simulink model "BESS_PV_WIND_STAGE2_R1_with_scopes"  (R2024b)
settings: Solver=VariableStepAuto  StartTime=0.0  StopTime=10.0  RelTol=1e-3
InitFcn:
  | run(fullfile(fileparts(get_param(bdroot,'FileName')),'..','scripts','init_bess_pv_wind_stage2_r1.m'));
undefined symbols (not defined in the file): Control, G, S1, S2, S21, W1
libraries: ee_lib x27, nesl_utility x23, fl_lib x10, simulink x5
(part 2 of 2)

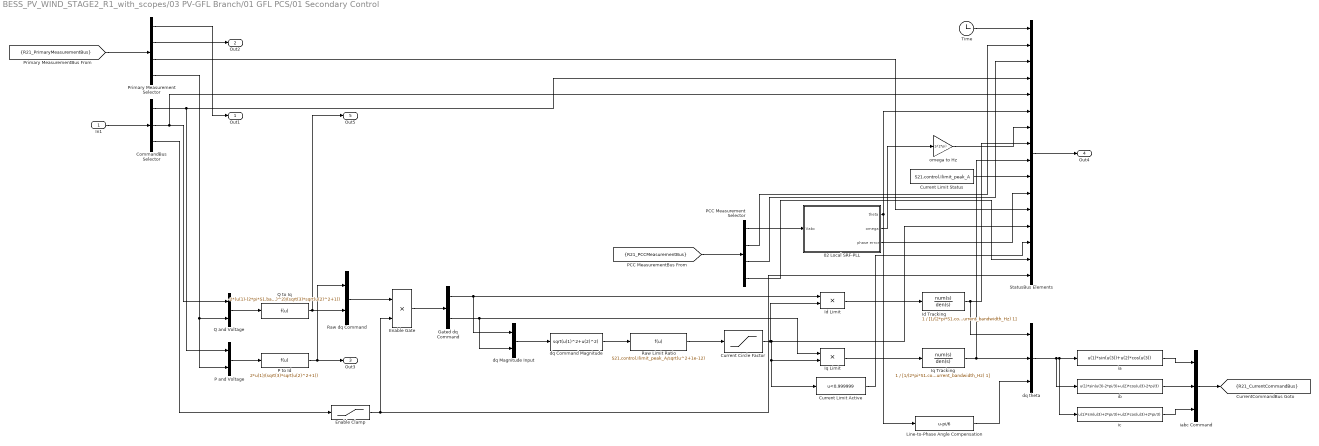
== system BESS_PV_WIND_STAGE2_R1_with_scopes/03 PV-GFL Branch/01 GFL PCS/01 Secondary Control ==
  In1 : Inport
  02 Local SRF-PLL : Subsystem
      settings: AttributesFormatString=|
      | local abc voltage only
      | wrapped phase-error PI
  CommandBus Selector : Demux  Outputs=3
  Current Circle Factor : Saturate  UpperLimit=1  LowerLimit=0
  Current Limit Active : Fcn  Expr=u<0.999999
  Current Limit Status : Constant  Value=S21.control.Ilimit_peak_A
  Enable Clamp : Saturate  UpperLimit=1  LowerLimit=0
  Enable Gate : Product  Inputs=**
  Gated dq Command : Demux  Outputs=2
  Id Limit : Product  Inputs=**
  Id Tracking : TransferFcn  Numerator=1  Denominator=[1/(2*pi*S1.control.current_bandwidth_Hz) 1]
  Iq Limit : Product  Inputs=**
  Iq Tracking : TransferFcn  Numerator=1  Denominator=[1/(2*pi*S1.control.current_bandwidth_Hz) 1]
  Line-to-Phase Angle Compensation : Fcn  Expr=u-pi/6
  P and Voltage : Mux  Inputs=2
  P to Id : Fcn  Expr=2*u(1)/(sqrt(3)*sqrt(u(2)^2+1))
  PCC Measurement Selector : Demux  Outputs=[3 1 1 1]
  Primary Measurement Selector : Demux  Outputs=[3 3 1 1]
  Q and Voltage : Mux  Inputs=2
  Q to Iq : Fcn  Expr=-2*(u(1)-(2*pi*S1.base.f_Hz*S1.filter.C_F/2)*u(2)^2)/(sqrt(3)*sqrt(u(2)^2+1))
  Raw Limit Ratio : Fcn  Expr=S21.control.Ilimit_peak_A/sqrt(u^2+1e-12)
  Raw dq Command : Mux  Inputs=2
  StatusBus Elements : Mux  Inputs=16
  Time : Clock
  dq Command Magnitude : Fcn  Expr=sqrt(u(1)^2+u(2)^2)
  dq Magnitude Input : Mux  Inputs=2
  dq theta : Mux  Inputs=3
  ia : Fcn  Expr=u(1)*sin(u(3))+u(2)*cos(u(3))
  iabc Command : Mux  Inputs=3
  ib : Fcn  Expr=u(1)*sin(u(3)-2*pi/3)+u(2)*cos(u(3)-2*pi/3)
  ic : Fcn  Expr=u(1)*sin(u(3)+2*pi/3)+u(2)*cos(u(3)+2*pi/3)
  omega to Hz : Gain  Gain=1/(2*pi)
  Out1 : Outport
  Out2 : Outport  Port=2
  Out3 : Outport  Port=3
  Out4 : Outport  Port=4
  Out5 : Outport  Port=5
  tag scope: R21_CurrentCommandBus=scoped
  wires:
  PCC Measurement Selector/4 -> StatusBus Elements/15
  Q and Voltage/1 -> Q to Iq/1
  Primary Measurement Selector/4 -> Q and Voltage/2, P and Voltage/2
  PCC Measurement Selector/3 -> StatusBus Elements/3
  Primary Measurement Selector/3 -> StatusBus Elements/12
  PCC Measurement Selector/2 -> StatusBus Elements/2
  Primary Measurement Selector/2 -> Out2/1
  PCC Measurement Selector/1 -> 02 Local SRF-PLL/1(Vabc)
  Primary Measurement Selector/1 -> Out1/1
  [R21_PCCMeasurementBus] -> PCC Measurement Selector/1
  Raw dq Command/1 -> Enable Gate/1
  [R21_PrimaryMeasurementBus] -> Primary Measurement Selector/1
  In1/1 -> CommandBus Selector/1
  CommandBus Selector/2 -> StatusBus Elements/5, Q and Voltage/1
  Current Limit Active/1 -> StatusBus Elements/14
  CommandBus Selector/1 -> P and Voltage/1, StatusBus Elements/4
  Current Limit Status/1 -> StatusBus Elements/10
  CommandBus Selector/3 -> Enable Clamp/1
  Id Tracking/1 -> StatusBus Elements/8, dq theta/1
  Gated dq Command/1 -> Id Limit/1, dq Magnitude Input/1
  P and Voltage/1 -> P to Id/1
  Q to Iq/1 -> Raw dq Command/2, Out5/1
  Gated dq Command/2 -> Iq Limit/1, dq Magnitude Input/2
  P to Id/1 -> Raw dq Command/1, Out3/1
  Enable Clamp/1 -> StatusBus Elements/16, Enable Gate/2
  Id Limit/1 -> Id Tracking/1
  Enable Gate/1 -> Gated dq Command/1
  dq Magnitude Input/1 -> dq Command Magnitude/1
  dq Command Magnitude/1 -> Raw Limit Ratio/1
  Raw Limit Ratio/1 -> Current Circle Factor/1
  Current Circle Factor/1 -> Current Limit Active/1, Iq Limit/2, StatusBus Elements/13, Id Limit/2
  02 Local SRF-PLL/1(theta) -> StatusBus Elements/6, Line-to-Phase Angle Compensation/1
  02 Local SRF-PLL/2(omega) -> omega to Hz/1
  02 Local SRF-PLL/3(phase error) -> StatusBus Elements/11
  Iq Limit/1 -> Iq Tracking/1
  Time/1 -> StatusBus Elements/1
  dq theta/1 -> ic/1, ia/1, ib/1
  omega to Hz/1 -> StatusBus Elements/7
  Iq Tracking/1 -> StatusBus Elements/9, dq theta/2
  Line-to-Phase Angle Compensation/1 -> dq theta/3
  StatusBus Elements/1 -> Out4/1
  ia/1 -> iabc Command/1
  ib/1 -> iabc Command/2
  ic/1 -> iabc Command/3
  iabc Command/1 -> [R21_CurrentCommandBus]

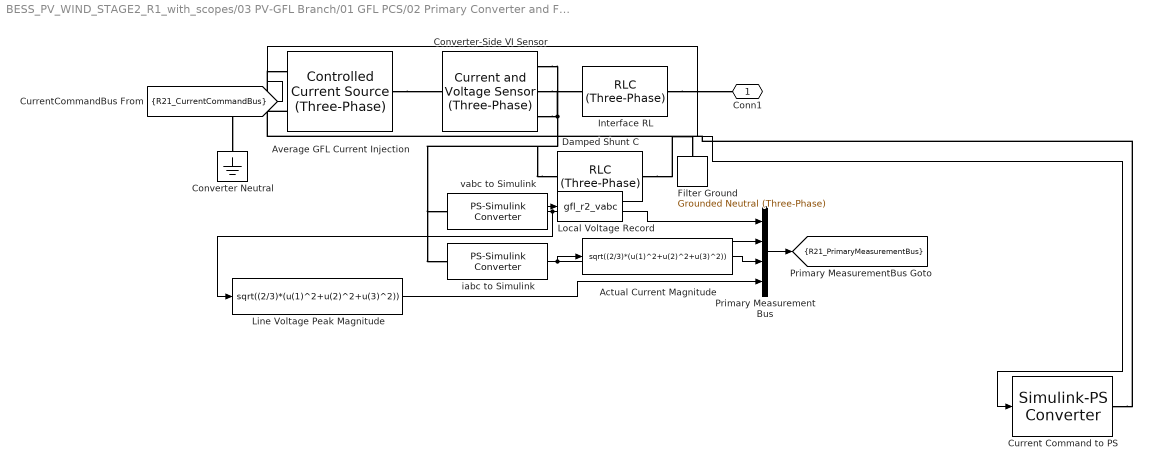
== system BESS_PV_WIND_STAGE2_R1_with_scopes/03 PV-GFL Branch/01 GFL PCS/02 Primary Converter and Filter ==
  Actual Current Magnitude : Fcn  Expr=sqrt((2/3)*(u(1)^2+u(2)^2+u(3)^2))
  Average GFL Current Injection : ee_lib/Sources/Controlled Current Source (Three-Phase)  port_option=ee.enum.threePhasePort.composite  input_option=ee.enum.inputType.instantaneous  FRated=S1.base.f_Hz Hz  G_parasitic=1e-6 1/Ohm
  Converter Neutral : fl_lib/Electrical/Electrical Elements/Electrical Reference
  Converter-Side VI Sensor : ee_lib/Sensors & Transducers/Current and Voltage Sensor (Three-Phase)  port_option=ee.enum.threePhasePort.composite  vMeasurementType=ee.enum.vmeasurement.ll  outputUnit=ee.enum.unit.si  SRated=100e6 A*V  VRated=24e3 V  I_specify=off  I_priority=None  I=[0, 0, 0] A  I_nominal_specify=off  I_nominal_value=1  I_nominal_unit=A  V_specify=off  V_priority=None  V=[0, 0, 0] V  V_nominal_specify=off  V_nominal_value=1  V_nominal_unit=V
  Current Command to PS : nesl_utility/Simulink-PS Converter  PhysicalDomain=network_engine_domain  SubClassName=ps_input  LeftPortType=input  RightPortType=output  PseudoPeriodic=off  Frequencies=[]  NoiseDistribution=none  NoiseParameters=[]  Unit=A  AffineConversion=off  FilteringAndDerivatives=zero  SimscapeFilterOrder=1  InputFilterTimeConstant=0.001  UdotUserProvided=0
  Damped Shunt C : ee_lib/Passive/RLC Assemblies/RLC (Three-Phase)  port_option=ee.enum.threePhasePort.composite  component_structure=ee.enum.rlc.structure.SeriesRC  R=S1.filter.Rd_ohm Ohm  L=1e-3 H  C=S1.filter.C_F F  R_parasitic=0 Ohm  G_parasitic=0 1/Ohm  IL_specify=off  IL_priority=High  IL=[0, 0, 0] A  IL_nominal_specify=off  IL_nominal_value=1  IL_nominal_unit=A  VC_specify=off  VC_priority=High  VC=[0, 0, 0] V  VC_nominal_specify=off  VC_nominal_value=1  VC_nominal_unit=V
  Filter Ground : ee_lib/Connectors & References/Grounded Neutral (Three-Phase)  port_option=ee.enum.threePhasePort.composite
  Interface RL : ee_lib/Passive/RLC Assemblies/RLC (Three-Phase)  port_option=ee.enum.threePhasePort.composite  component_structure=ee.enum.rlc.structure.R  R=S1.filter.R1_ohm+S1.filter.R2_ohm Ohm  L=1e-3 H  C=1e-6 F  R_parasitic=0 Ohm  G_parasitic=0 1/Ohm  IL_specify=off  IL_priority=High  IL=[0, 0, 0] A  IL_nominal_specify=off  IL_nominal_value=1  IL_nominal_unit=A  VC_specify=off  VC_priority=High  VC=[0, 0, 0] V  VC_nominal_specify=off  VC_nominal_value=1  VC_nominal_unit=V
  Line Voltage Peak Magnitude : Fcn  Expr=sqrt((2/3)*(u(1)^2+u(2)^2+u(3)^2))
  Local Voltage Record : ToWorkspace  VariableName=gfl_r2_vabc  SampleTime=-1
  Primary MeasurementBus : Mux
  iabc to Simulink : nesl_utility/PS-Simulink Converter  PhysicalDomain=network_engine_domain  SubClassName=ps_output  LeftPortType=input  RightPortType=output  PseudoPeriodic=off  Frequencies=[]  VectorFormat=inherit  Unit=A  AffineConversion=off
  vabc to Simulink : nesl_utility/PS-Simulink Converter  PhysicalDomain=network_engine_domain  SubClassName=ps_output  LeftPortType=input  RightPortType=output  PseudoPeriodic=off  Frequencies=[]  VectorFormat=inherit  Unit=V  AffineConversion=off
  Conn1 : PMIOPort  Side=Right
  tag scope: R21_PrimaryMeasurementBus=scoped
  wires:
  iabc to Simulink/1 -> Primary MeasurementBus/2, Actual Current Magnitude/1
  vabc to Simulink/1 -> Primary MeasurementBus/1, Line Voltage Peak Magnitude/1, Local Voltage Record/1
  [R21_CurrentCommandBus] -> Current Command to PS/1
  Primary MeasurementBus/1 -> [R21_PrimaryMeasurementBus]
  Actual Current Magnitude/1 -> Primary MeasurementBus/3
  Line Voltage Peak Magnitude/1 -> Primary MeasurementBus/4
  connections:
  Damped Shunt C/LConn1 -- Converter-Side VI Sensor/RConn3 -- Interface RL/LConn1
  Current Command to PS/RConn1 -- Average GFL Current Injection/LConn1
  Converter-Side VI Sensor/RConn1 -- vabc to Simulink/LConn1
  Average GFL Current Injection/LConn2 -- Converter Neutral/LConn1
  Interface RL/RConn1 -- Conn1/RConn1
  Converter-Side VI Sensor/RConn2 -- iabc to Simulink/LConn1
  Damped Shunt C/RConn1 -- Filter Ground/LConn1
  Average GFL Current Injection/RConn1 -- Converter-Side VI Sensor/LConn1

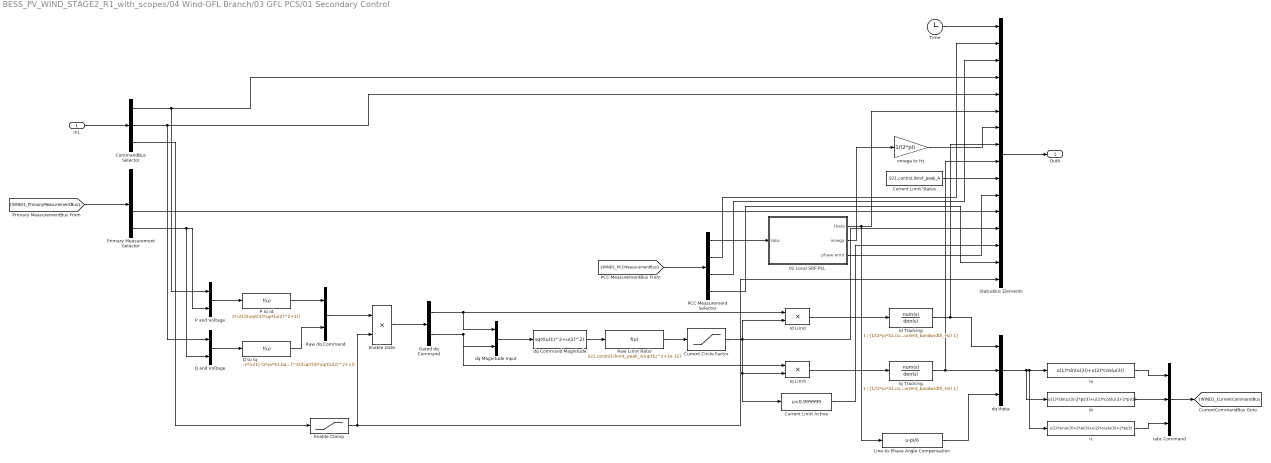
== system BESS_PV_WIND_STAGE2_R1_with_scopes/04 Wind-GFL Branch/03 GFL PCS/01 Secondary Control ==
  In1 : Inport
  02 Local SRF-PLL : Subsystem
      settings: AttributesFormatString=|
      | local abc voltage only
      | wrapped phase-error PI
  CommandBus Selector : Demux  Outputs=3
  Current Circle Factor : Saturate  UpperLimit=1  LowerLimit=0
  Current Limit Active : Fcn  Expr=u<0.999999
  Current Limit Status : Constant  Value=S21.control.Ilimit_peak_A
  Enable Clamp : Saturate  UpperLimit=1  LowerLimit=0
  Enable Gate : Product  Inputs=**
  Gated dq Command : Demux  Outputs=2
  Id Limit : Product  Inputs=**
  Id Tracking : TransferFcn  Numerator=1  Denominator=[1/(2*pi*S1.control.current_bandwidth_Hz) 1]
  Iq Limit : Product  Inputs=**
  Iq Tracking : TransferFcn  Numerator=1  Denominator=[1/(2*pi*S1.control.current_bandwidth_Hz) 1]
  Line-to-Phase Angle Compensation : Fcn  Expr=u-pi/6
  P and Voltage : Mux  Inputs=2
  P to Id : Fcn  Expr=2*u(1)/(sqrt(3)*sqrt(u(2)^2+1))
  PCC Measurement Selector : Demux  Outputs=[3 1 1 1]
  Primary Measurement Selector : Demux  Outputs=[3 3 1 1]
  Q and Voltage : Mux  Inputs=2
  Q to Iq : Fcn  Expr=-2*(u(1)-(2*pi*S1.base.f_Hz*S1.filter.C_F/2)*u(2)^2)/(sqrt(3)*sqrt(u(2)^2+1))
  Raw Limit Ratio : Fcn  Expr=S21.control.Ilimit_peak_A/sqrt(u^2+1e-12)
  Raw dq Command : Mux  Inputs=2
  StatusBus Elements : Mux  Inputs=16
  Time : Clock
  dq Command Magnitude : Fcn  Expr=sqrt(u(1)^2+u(2)^2)
  dq Magnitude Input : Mux  Inputs=2
  dq theta : Mux  Inputs=3
  ia : Fcn  Expr=u(1)*sin(u(3))+u(2)*cos(u(3))
  iabc Command : Mux  Inputs=3
  ib : Fcn  Expr=u(1)*sin(u(3)-2*pi/3)+u(2)*cos(u(3)-2*pi/3)
  ic : Fcn  Expr=u(1)*sin(u(3)+2*pi/3)+u(2)*cos(u(3)+2*pi/3)
  omega to Hz : Gain  Gain=1/(2*pi)
  Out4 : Outport
  tag scope: WIND1_CurrentCommandBus=scoped
  wires:
  In1/1 -> CommandBus Selector/1
  Primary Measurement Selector/4 -> P and Voltage/2, Q and Voltage/2
  Enable Clamp/1 -> StatusBus Elements/16, Enable Gate/2
  P to Id/1 -> Raw dq Command/1
  [WIND1_PrimaryMeasurementBus] -> Primary Measurement Selector/1
  CommandBus Selector/3 -> Enable Clamp/1
  CommandBus Selector/1 -> StatusBus Elements/4, P and Voltage/1
  CommandBus Selector/2 -> StatusBus Elements/5, Q and Voltage/1
  Id Tracking/1 -> dq theta/1, StatusBus Elements/8
  P and Voltage/1 -> P to Id/1
  Primary Measurement Selector/3 -> StatusBus Elements/12
  Q and Voltage/1 -> Q to Iq/1
  iabc Command/1 -> [WIND1_CurrentCommandBus]
  Q to Iq/1 -> Raw dq Command/2
  Raw dq Command/1 -> Enable Gate/1
  PCC Measurement Selector/2 -> StatusBus Elements/2
  Enable Gate/1 -> Gated dq Command/1
  Gated dq Command/1 -> Id Limit/1, dq Magnitude Input/1
  [WIND1_PCCMeasurementBus] -> PCC Measurement Selector/1
  Gated dq Command/2 -> Iq Limit/1, dq Magnitude Input/2
  dq Magnitude Input/1 -> dq Command Magnitude/1
  dq Command Magnitude/1 -> Raw Limit Ratio/1
  Raw Limit Ratio/1 -> Current Circle Factor/1
  Iq Limit/1 -> Iq Tracking/1
  PCC Measurement Selector/1 -> 02 Local SRF-PLL/1(Vabc)
  PCC Measurement Selector/3 -> StatusBus Elements/3
  Iq Tracking/1 -> StatusBus Elements/9, dq theta/2
  Current Circle Factor/1 -> Current Limit Active/1, Iq Limit/2, StatusBus Elements/13, Id Limit/2
  PCC Measurement Selector/4 -> StatusBus Elements/15
  02 Local SRF-PLL/1(theta) -> StatusBus Elements/6, Line-to-Phase Angle Compensation/1
  02 Local SRF-PLL/2(omega) -> omega to Hz/1
  02 Local SRF-PLL/3(phase error) -> StatusBus Elements/11
  Id Limit/1 -> Id Tracking/1
  Line-to-Phase Angle Compensation/1 -> dq theta/3
  Current Limit Active/1 -> StatusBus Elements/14
  Time/1 -> StatusBus Elements/1
  dq theta/1 -> ia/1, ic/1, ib/1
  omega to Hz/1 -> StatusBus Elements/7
  Current Limit Status/1 -> StatusBus Elements/10
  StatusBus Elements/1 -> Out4/1
  ia/1 -> iabc Command/1
  ib/1 -> iabc Command/2
  ic/1 -> iabc Command/3

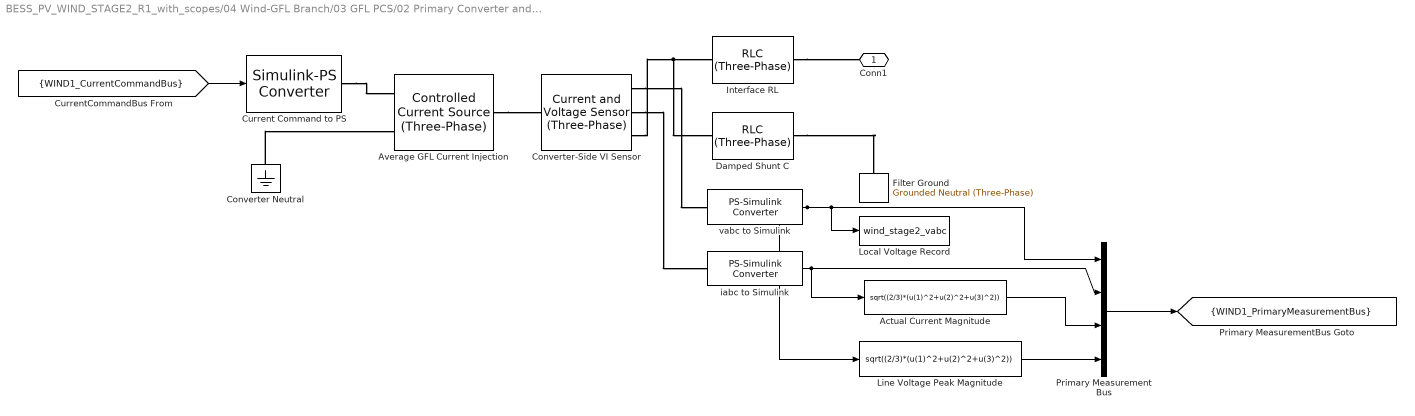
== system BESS_PV_WIND_STAGE2_R1_with_scopes/04 Wind-GFL Branch/03 GFL PCS/02 Primary Converter and Filter ==
  Actual Current Magnitude : Fcn  Expr=sqrt((2/3)*(u(1)^2+u(2)^2+u(3)^2))
  Average GFL Current Injection : ee_lib/Sources/Controlled Current Source (Three-Phase)  port_option=ee.enum.threePhasePort.composite  input_option=ee.enum.inputType.instantaneous  FRated=S1.base.f_Hz Hz  G_parasitic=1e-6 1/Ohm
  Converter Neutral : fl_lib/Electrical/Electrical Elements/Electrical Reference
  Converter-Side VI Sensor : ee_lib/Sensors & Transducers/Current and Voltage Sensor (Three-Phase)  port_option=ee.enum.threePhasePort.composite  vMeasurementType=ee.enum.vmeasurement.ll  outputUnit=ee.enum.unit.si  SRated=100e6 A*V  VRated=24e3 V  I_specify=off  I_priority=None  I=[0, 0, 0] A  I_nominal_specify=off  I_nominal_value=1  I_nominal_unit=A  V_specify=off  V_priority=None  V=[0, 0, 0] V  V_nominal_specify=off  V_nominal_value=1  V_nominal_unit=V
  Current Command to PS : nesl_utility/Simulink-PS Converter  PhysicalDomain=network_engine_domain  SubClassName=ps_input  LeftPortType=input  RightPortType=output  PseudoPeriodic=off  Frequencies=[]  NoiseDistribution=none  NoiseParameters=[]  Unit=A  AffineConversion=off  FilteringAndDerivatives=zero  SimscapeFilterOrder=1  InputFilterTimeConstant=0.001  UdotUserProvided=0
  Damped Shunt C : ee_lib/Passive/RLC Assemblies/RLC (Three-Phase)  port_option=ee.enum.threePhasePort.composite  component_structure=ee.enum.rlc.structure.SeriesRC  R=S1.filter.Rd_ohm Ohm  L=1e-3 H  C=S1.filter.C_F F  R_parasitic=0 Ohm  G_parasitic=0 1/Ohm  IL_specify=off  IL_priority=High  IL=[0, 0, 0] A  IL_nominal_specify=off  IL_nominal_value=1  IL_nominal_unit=A  VC_specify=off  VC_priority=High  VC=[0, 0, 0] V  VC_nominal_specify=off  VC_nominal_value=1  VC_nominal_unit=V
  Filter Ground : ee_lib/Connectors & References/Grounded Neutral (Three-Phase)  port_option=ee.enum.threePhasePort.composite
  Interface RL : ee_lib/Passive/RLC Assemblies/RLC (Three-Phase)  port_option=ee.enum.threePhasePort.composite  component_structure=ee.enum.rlc.structure.R  R=S1.filter.R1_ohm+S1.filter.R2_ohm Ohm  L=1e-3 H  C=1e-6 F  R_parasitic=0 Ohm  G_parasitic=0 1/Ohm  IL_specify=off  IL_priority=High  IL=[0, 0, 0] A  IL_nominal_specify=off  IL_nominal_value=1  IL_nominal_unit=A  VC_specify=off  VC_priority=High  VC=[0, 0, 0] V  VC_nominal_specify=off  VC_nominal_value=1  VC_nominal_unit=V
  Line Voltage Peak Magnitude : Fcn  Expr=sqrt((2/3)*(u(1)^2+u(2)^2+u(3)^2))
  Local Voltage Record : ToWorkspace  VariableName=wind_stage2_vabc  SampleTime=-1
  Primary MeasurementBus : Mux
  iabc to Simulink : nesl_utility/PS-Simulink Converter  PhysicalDomain=network_engine_domain  SubClassName=ps_output  LeftPortType=input  RightPortType=output  PseudoPeriodic=off  Frequencies=[]  VectorFormat=inherit  Unit=A  AffineConversion=off
  vabc to Simulink : nesl_utility/PS-Simulink Converter  PhysicalDomain=network_engine_domain  SubClassName=ps_output  LeftPortType=input  RightPortType=output  PseudoPeriodic=off  Frequencies=[]  VectorFormat=inherit  Unit=V  AffineConversion=off
  Conn1 : PMIOPort  Side=Right
  tag scope: WIND1_PrimaryMeasurementBus=scoped
  wires:
  vabc to Simulink/1 -> Line Voltage Peak Magnitude/1, Primary MeasurementBus/1, Local Voltage Record/1
  Actual Current Magnitude/1 -> Primary MeasurementBus/3
  [WIND1_CurrentCommandBus] -> Current Command to PS/1
  Line Voltage Peak Magnitude/1 -> Primary MeasurementBus/4
  Primary MeasurementBus/1 -> [WIND1_PrimaryMeasurementBus]
  iabc to Simulink/1 -> Primary MeasurementBus/2, Actual Current Magnitude/1
  connections:
  Interface RL/RConn1 -- Conn1/RConn1
  Converter-Side VI Sensor/RConn2 -- iabc to Simulink/LConn1
  Average GFL Current Injection/RConn1 -- Converter-Side VI Sensor/LConn1
  Converter Neutral/LConn1 -- Average GFL Current Injection/LConn2
  Current Command to PS/RConn1 -- Average GFL Current Injection/LConn1
  Converter-Side VI Sensor/RConn3 -- Interface RL/LConn1 -- Damped Shunt C/LConn1
  Converter-Side VI Sensor/RConn1 -- vabc to Simulink/LConn1
  Damped Shunt C/RConn1 -- Filter Ground/LConn1

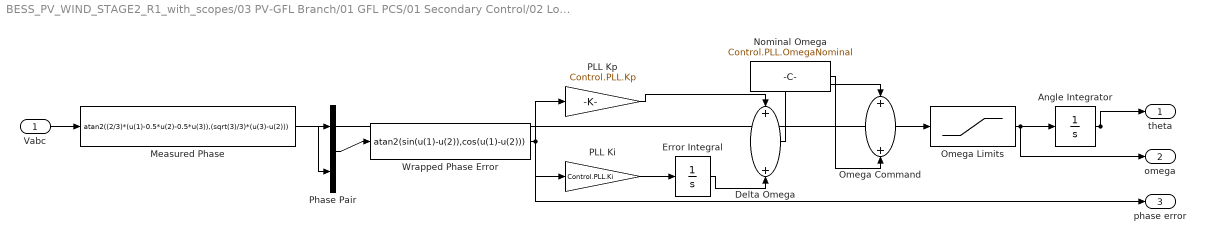
== system BESS_PV_WIND_STAGE2_R1_with_scopes/03 PV-GFL Branch/01 GFL PCS/01 Secondary Control/02 Local SRF-PLL ==
  Vabc : Inport
  Angle Integrator : Integrator  InitialCondition=Control.PLL.Theta0
  Delta Omega : Sum
  Error Integral : Integrator
  Measured Phase : Fcn  Expr=atan2((2/3)*(u(1)-0.5*u(2)-0.5*u(3)),(sqrt(3)/3)*(u(3)-u(2)))
  Nominal Omega : Constant  Value=Control.PLL.OmegaNominal
  Omega Command : Sum
  Omega Limits : Saturate  UpperLimit=Control.PLL.OmegaMax  LowerLimit=Control.PLL.OmegaMin
  PLL Ki : Gain  Gain=Control.PLL.Ki
  PLL Kp : Gain  Gain=Control.PLL.Kp
  Phase Pair : Mux  Inputs=2
  Wrapped Phase Error : Fcn  Expr=atan2(sin(u(1)-u(2)),cos(u(1)-u(2)))
  theta : Outport
  omega : Outport  Port=2
  phase error : Outport  Port=3
  wires:
  Omega Limits/1 -> omega/1, Angle Integrator/1
  Omega Command/1 -> Omega Limits/1
  Nominal Omega/1 -> Omega Command/2
  Delta Omega/1 -> Omega Command/1
  Error Integral/1 -> Delta Omega/2
  PLL Kp/1 -> Delta Omega/1
  PLL Ki/1 -> Error Integral/1
  Wrapped Phase Error/1 -> phase error/1, PLL Ki/1, PLL Kp/1
  Phase Pair/1 -> Wrapped Phase Error/1
  Angle Integrator/1 -> theta/1, Phase Pair/2
  Measured Phase/1 -> Phase Pair/1
  Vabc/1 -> Measured Phase/1

== system BESS_PV_WIND_STAGE2_R1_with_scopes/04 Wind-GFL Branch/03 GFL PCS/01 Secondary Control/02 Local SRF-PLL ==
  Vabc : Inport
  Angle Integrator : Integrator  InitialCondition=Control.PLL.Theta0
  Delta Omega : Sum
  Error Integral : Integrator
  Measured Phase : Fcn  Expr=atan2((2/3)*(u(1)-0.5*u(2)-0.5*u(3)),(sqrt(3)/3)*(u(3)-u(2)))
  Nominal Omega : Constant  Value=Control.PLL.OmegaNominal
  Omega Command : Sum
  Omega Limits : Saturate  UpperLimit=Control.PLL.OmegaMax  LowerLimit=Control.PLL.OmegaMin  ZeroCross=off
  PLL Ki : Gain  Gain=Control.PLL.Ki
  PLL Kp : Gain  Gain=Control.PLL.Kp
  Phase Pair : Mux  Inputs=2
  Wrapped Phase Error : Fcn  Expr=atan2(sin(u(1)-u(2)),cos(u(1)-u(2)))
  theta : Outport
  omega : Outport  Port=2
  phase error : Outport  Port=3
  wires:
  Omega Limits/1 -> omega/1, Angle Integrator/1
  Omega Command/1 -> Omega Limits/1
  Nominal Omega/1 -> Omega Command/2
  Delta Omega/1 -> Omega Command/1
  Error Integral/1 -> Delta Omega/2
  PLL Kp/1 -> Delta Omega/1
  PLL Ki/1 -> Error Integral/1
  Wrapped Phase Error/1 -> phase error/1, PLL Ki/1, PLL Kp/1
  Phase Pair/1 -> Wrapped Phase Error/1
  Angle Integrator/1 -> theta/1, Phase Pair/2
  Measured Phase/1 -> Phase Pair/1
  Vabc/1 -> Measured Phase/1
